simulink model "reinforcemen_model4"  (R2023b)
settings: Solver=FixedStepAuto  StartTime=0.0  StopTime=17  FixedStep=0.05  RelTol=1e-3  EnableMultiTasking=on
model workspace (MAT data in the model file):
  adjected_goal = 0
libraries: simulink x7, rllib x5
settings Model: SimulationMode=accelerator  ExtModeTrigDuration=2  Creator=MSI PC  LastModifiedBy=Yuk
settings SolverCC: AutoInsertRateTranBlk=on
settings OptimizationCC: DefaultParameterBehavior=Inlined  EnhancedBackFolding=on  PassReuseOutputArgsAs=Individual arguments  ZeroExternalMemoryAtStartup=off  ZeroInternalMemoryAtStartup=off  MaxStackSize=64  OptimizeBlockOrder=speed  DifferentSizesBufferReuse=on  OptimizationCustomize=off  EfficientTunableParamExpr=on
settings DebuggingCC: ParameterTunabilityLossMsg=error  UnconnectedInputMsg=warning  UnconnectedOutputMsg=warning  UnconnectedLineMsg=warning
settings HardwareCC: ProdBitPerPointer=32  ProdBitPerSizeT=32  ProdBitPerPtrDiffT=32  ProdLargestAtomicInteger=Long  ProdLargestAtomicFloat=Double  ProdWordSize=32  ProdHWDeviceType=ARM Compatible->ARM Cortex
settings ModelReferenceCC: EnableRefExpFcnMdlSchedulingChecks=on
settings SFSimCC: MATLABDynamicMemAlloc=off
settings RTWCC: Description=Embedded Coder  SystemTargetFile=ert.tlc  TemplateMakefile=ert_default_tmf  BuildConfiguration=Faster Runs  DLArmComputeVersion=19.05
settings CodeAppCC: ForceParamTrailComments=on  IgnoreCustomStorageClasses=off  OperatorAnnotations=on  SimulinkDataObjDesc=on  SFDataObjDesc=on  InsertBlockDesc=on
settings ERTTargetCC: SupportContinuousTime=on  SupportVariableSizeSignals=on  ExtModeTransport=3  ExtModeStaticAlloc=on  ExtModeAutomaticAllocSize=off  ExtModeStaticAllocSize=8192  ExtModeMexFile=ext_xcp  ExtModeIntrfLevel=Level2 - Open  ERTCustomFileTemplate=example_file_process.tlc

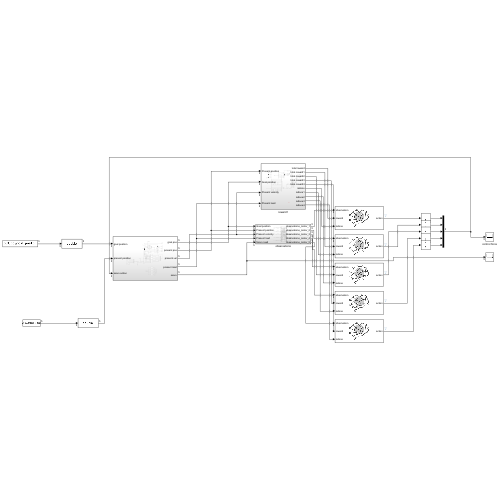
[thumbnail: Simulink's stored preview of the top-level diagram]
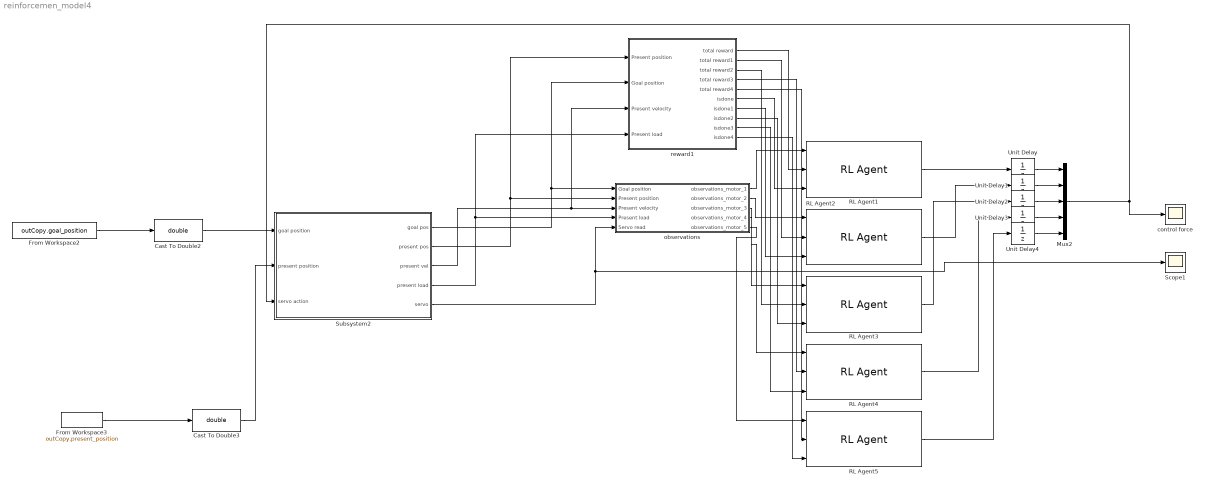
== system reinforcemen_model4 ==
  Cast To Double2 : DataTypeConversion  OutDataTypeStr=double  SaturateOnIntegerOverflow=off  RndMeth=Floor
  Cast To Double3 : DataTypeConversion  OutDataTypeStr=double  SaturateOnIntegerOverflow=off  RndMeth=Floor
  From Workspace2 : FromWorkspace  VariableName=outCopy.goal_position
  From Workspace3 : FromWorkspace  VariableName=outCopy.present_position
  Mux2 : Mux  Inputs=5
  RL Agent1 : rllib/RL Agent  Agent=agentA  ExternalActionAsInput=off  ProvideLastAction=off  ProvideCumRwd=off  TreatAsDirectFeedthrough=on  UseStrictObservationDataTypes=off
  RL Agent2 : rllib/RL Agent  Agent=agentB  ExternalActionAsInput=off  ProvideLastAction=off  ProvideCumRwd=off  TreatAsDirectFeedthrough=on  UseStrictObservationDataTypes=off
  RL Agent3 : rllib/RL Agent  Agent=agentC  ExternalActionAsInput=off  ProvideLastAction=off  ProvideCumRwd=off  TreatAsDirectFeedthrough=on  UseStrictObservationDataTypes=off
  RL Agent4 : rllib/RL Agent  Agent=agentD  ExternalActionAsInput=off  ProvideLastAction=off  ProvideCumRwd=off  TreatAsDirectFeedthrough=on  UseStrictObservationDataTypes=off
  RL Agent5 : rllib/RL Agent  Agent=agentE  ExternalActionAsInput=off  ProvideLastAction=off  ProvideCumRwd=off  TreatAsDirectFeedthrough=on  UseStrictObservationDataTypes=off
  Scope1 : Scope
  Subsystem2 : Subsystem
  Unit Delay : UnitDelay  SampleTime=-1  HasFrameUpgradeWarning=on
  Unit Delay{1..4} (4 alike) : UnitDelay  InitialCondition=180  SampleTime=-1  HasFrameUpgradeWarning=on
  control force : Scope
  observations : Subsystem
  reward1 : Subsystem
  wires:
  Subsystem2/1(goal pos) -> reward1/2(Goal position), observations/1(Goal position)
  RL Agent3/1 -> Unit Delay2/1
  RL Agent2/1 -> Unit Delay1/1
  RL Agent4/1 -> Unit Delay3/1
  RL Agent5/1 -> Unit Delay4/1
  observations/1(observations_motor_1) -> RL Agent1/1
  observations/2(observations_motor_2) -> RL Agent2/1
  observations/3(observations_motor_3) -> RL Agent3/1
  observations/4(observations_motor_4) -> RL Agent4/1
  observations/5(observations_motor_5) -> RL Agent5/1
  Subsystem2/5(servo) -> Scope1/1, observations/5(Servo read)
  reward1/1(total reward) -> RL Agent1/2
  reward1/2(total reward1) -> RL Agent2/2
  reward1/3(total reward2) -> RL Agent3/2
  reward1/4(total reward3) -> RL Agent4/2
  reward1/5(total reward4) -> RL Agent5/2
  reward1/6(isdone) -> RL Agent1/3
  reward1/7(isdone1) -> RL Agent2/3
  reward1/8(isdone2) -> RL Agent3/3
  reward1/9(isdone3) -> RL Agent4/3
  reward1/10(isdone4) -> RL Agent5/3
  Subsystem2/2(present pos) -> reward1/1(Present position), observations/2(Present position)
  Subsystem2/4(present load) -> reward1/4(Present load), observations/4(Present load)
  Subsystem2/3(present vel) -> reward1/3(Present velocity), observations/3(Present velocity)
  Mux2/1 -> Subsystem2/3(servo action), control force/1
  RL Agent1/1 -> Unit Delay/1
  Cast To Double2/1 -> Subsystem2/1(goal position)
  From Workspace2/1 -> Cast To Double2/1
  Cast To Double3/1 -> Subsystem2/2(present position)
  From Workspace3/1 -> Cast To Double3/1
  Unit Delay/1 -> Mux2/1
  Unit Delay1/1 -> Mux2/2
  Unit Delay2/1 -> Mux2/3
  Unit Delay3/1 -> Mux2/4
  Unit Delay4/1 -> Mux2/5

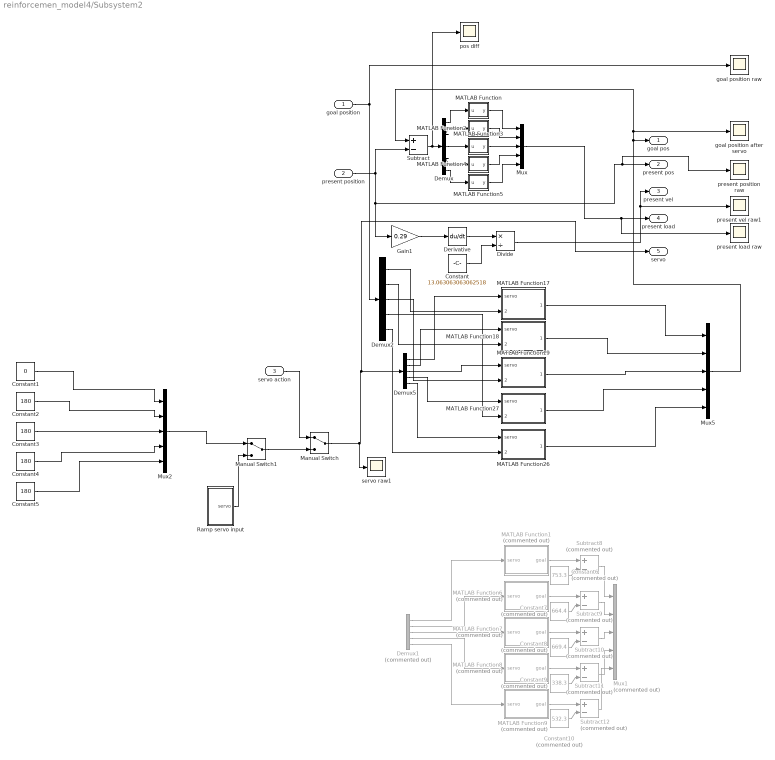
== system reinforcemen_model4/Subsystem2 ==
  goal position : Inport
  present position : Inport  Port=2
  servo action : Inport  Port=3
  Constant : Constant  Value=13.063063063062518
  Constant1 : Constant  Value=0
  Constant10 : Constant  Commented=on  Value=532.3
  Constant{2..5} (4 alike) : Constant  Value=180
  Constant6 : Constant  Commented=on  Value=753.3
  Constant7 : Constant  Commented=on  Value=664.4
  Constant8 : Constant  Commented=on  Value=669.4
  Constant9 : Constant  Commented=on  Value=338.3
  Demux : Demux  Outputs=5
  Demux1 : Demux  Commented=on  Outputs=5
  Demux2 : Demux  Outputs=5
  Demux5 : Demux  Outputs=5
  Derivative : Derivative
  Divide : Product  Inputs=*/
  Gain1 : Gain  Gain=0.29
  MATLAB Function : MATLAB Function  TreatAsAtomicUnit=on
  MATLAB Function1 : MATLAB Function  Commented=on  TreatAsAtomicUnit=on
  MATLAB Function17 : MATLAB Function  TreatAsAtomicUnit=on
  MATLAB Function18 : MATLAB Function  TreatAsAtomicUnit=on
  MATLAB Function19 : MATLAB Function  TreatAsAtomicUnit=on
  MATLAB Function2 : MATLAB Function  TreatAsAtomicUnit=on
  MATLAB Function26 : MATLAB Function  TreatAsAtomicUnit=on
  MATLAB Function27 : MATLAB Function  TreatAsAtomicUnit=on
  MATLAB Function3 : MATLAB Function  TreatAsAtomicUnit=on
  MATLAB Function4 : MATLAB Function  TreatAsAtomicUnit=on
  MATLAB Function5 : MATLAB Function  TreatAsAtomicUnit=on
  MATLAB Function6 : MATLAB Function  Commented=on  TreatAsAtomicUnit=on
  MATLAB Function7 : MATLAB Function  Commented=on  TreatAsAtomicUnit=on
  MATLAB Function8 : MATLAB Function  Commented=on  TreatAsAtomicUnit=on
  MATLAB Function9 : MATLAB Function  Commented=on  TreatAsAtomicUnit=on
  Manual Switch : ManualSwitch
  Manual Switch1 : ManualSwitch
  Mux : Mux  Inputs=5
  Mux1 : Mux  Commented=on  Inputs=5
  Mux2 : Mux  Inputs=5
  Mux5 : Mux  Inputs=5
  Ramp servo input : Subsystem
  Subtract : Sum  Inputs=+-
  Subtract{8..12} (5 alike) : Sum  Commented=on  Inputs=+-
  goal position after servo : Scope
  goal position raw : Scope
  pos diff : Scope
  present load raw : Scope
  present position raw : Scope
  present vel raw1 : Scope
  servo raw1 : Scope
  goal pos : Outport
  present pos : Outport  Port=2
  present vel : Outport  Port=3
  present load : Outport  Port=4
  servo : Outport  Port=5
  wires:
  goal position/1 -> goal position raw/1, Demux2/1
  present position/1 -> Subtract/2, Gain1/1, present position raw/1, present pos/1
  Demux/2 -> MATLAB Function2/1(u)
  MATLAB Function3/1(y) -> Mux/3
  Mux/1 -> present load raw/1, present load/1
  MATLAB Function/1(y) -> Mux/1
  MATLAB Function5/1(y) -> Mux/5
  MATLAB Function4/1(y) -> Mux/4
  Demux/4 -> MATLAB Function4/1(u)
  Demux/3 -> MATLAB Function3/1(u)
  Demux/1 -> MATLAB Function/1(u)
  Demux/5 -> MATLAB Function5/1(u)
  MATLAB Function2/1(y) -> Mux/2
  Constant/1 -> Divide/2
  Gain1/1 -> Derivative/1
  Derivative/1 -> Divide/1
  Divide/1 -> present vel raw1/1, present vel/1
  Demux5/3 -> MATLAB Function19/1(servo)
  Demux5/2 -> MATLAB Function18/1(servo)
  Demux5/1 -> MATLAB Function17/1(servo)
  Demux5/5 -> MATLAB Function26/1(servo)
  Demux5/4 -> MATLAB Function27/1(servo)
  Mux5/1 -> Subtract/1, goal position after servo/1, goal pos/1
  MATLAB Function9/1(goal) -> Subtract12/1
  Constant10/1 -> Subtract12/2
  Constant9/1 -> Subtract11/2
  MATLAB Function8/1(goal) -> Subtract11/1
  Subtract12/1 -> Mux1/5
  Subtract11/1 -> Mux1/4
  Subtract10/1 -> Mux1/3
  MATLAB Function7/1(goal) -> Subtract10/1
  Constant8/1 -> Subtract10/2
  Constant7/1 -> Subtract9/2
  Subtract9/1 -> Mux1/2
  Subtract8/1 -> Mux1/1
  MATLAB Function6/1(goal) -> Subtract9/1
  Constant6/1 -> Subtract8/2
  MATLAB Function1/1(goal) -> Subtract8/1
  Demux1/4 -> MATLAB Function8/1(servo)
  Demux1/5 -> MATLAB Function9/1(servo)
  Demux1/1 -> MATLAB Function1/1(servo)
  Demux1/2 -> MATLAB Function6/1(servo)
  Demux1/3 -> MATLAB Function7/1(servo)
  MATLAB Function17/1(adjected_goal) -> Mux5/1
  MATLAB Function18/1(adjected_goal) -> Mux5/2
  MATLAB Function19/1(adjected_goal) -> Mux5/3
  MATLAB Function27/1(adjected_goal) -> Mux5/4
  MATLAB Function26/1(adjected_goal) -> Mux5/5
  Constant2/1 -> Mux2/2
  Constant5/1 -> Mux2/5
  Constant1/1 -> Mux2/1
  Constant3/1 -> Mux2/3
  Constant4/1 -> Mux2/4
  Demux2/1 -> MATLAB Function17/2(init_goal)
  Demux2/2 -> MATLAB Function18/2(init_goal)
  Demux2/3 -> MATLAB Function19/2(init_goal)
  Demux2/4 -> MATLAB Function27/2(init_goal)
  Demux2/5 -> MATLAB Function26/2(init_goal)
  Manual Switch/1 -> servo raw1/1, servo/1, Demux5/1
  servo action/1 -> Manual Switch/1
  Manual Switch1/1 -> Manual Switch/2
  Mux2/1 -> Manual Switch1/1
  Ramp servo input/1(servo) -> Manual Switch1/2
  Subtract/1 -> pos diff/1, Demux/1

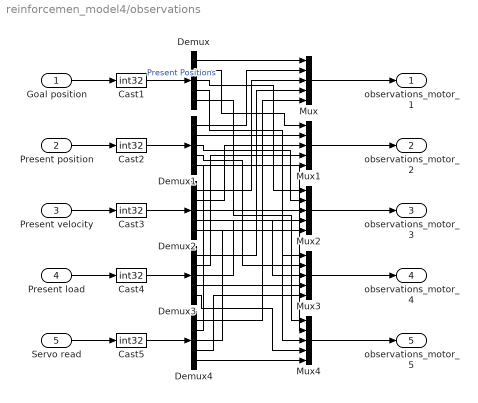
== system reinforcemen_model4/observations ==
  Goal position : Inport
  Present position : Inport  Port=2
  Present velocity : Inport  Port=3
  Present load : Inport  Port=4
  Servo read : Inport  Port=5
  Cast{1..5} (5 alike) : DataTypeConversion  OutDataTypeStr=int32  SaturateOnIntegerOverflow=off  RndMeth=Floor
  Demux{,1..4} (5 alike) : Demux  Outputs=5
  Mux{,1..4} (5 alike) : Mux  Inputs=5
  observations_motor_1 : Outport
  observations_motor_2 : Outport  Port=2
  observations_motor_3 : Outport  Port=3
  observations_motor_4 : Outport  Port=4
  observations_motor_5 : Outport  Port=5
  wires:
  Goal position/1 -> Cast1/1
  Present position/1 -> Cast2/1
  Present velocity/1 -> Cast3/1
  Present load/1 -> Cast4/1
  Servo read/1 -> Cast5/1
  Demux/1 -> Mux/1
  Demux1/1 -> Mux/2
  Demux2/1 -> Mux/3
  Demux3/1 -> Mux/4
  Demux4/1 -> Mux/5
  Demux/2 -> Mux1/1
  Demux1/2 -> Mux1/2
  Demux2/2 -> Mux1/3
  Demux3/2 -> Mux1/4
  Demux4/2 -> Mux1/5
  Demux/3 -> Mux2/1
  Demux1/3 -> Mux2/2
  Demux2/3 -> Mux2/3
  Demux3/3 -> Mux2/4
  Demux4/3 -> Mux2/5
  Demux/4 -> Mux3/1
  Demux1/4 -> Mux3/2
  Demux2/4 -> Mux3/3
  Demux3/4 -> Mux3/4
  Demux4/4 -> Mux3/5
  Demux/5 -> Mux4/1
  Demux1/5 -> Mux4/2
  Demux2/5 -> Mux4/3
  Demux3/5 -> Mux4/4
  Demux4/5 -> Mux4/5
  Mux/1 -> observations_motor_1/1
  Mux1/1 -> observations_motor_2/1
  Mux2/1 -> observations_motor_3/1
  Mux3/1 -> observations_motor_4/1
  Mux4/1 -> observations_motor_5/1
  Cast2/1 -> Demux1/1
  Cast3/1 -> Demux2/1
  Cast4/1 -> Demux3/1
  Cast5/1 -> Demux4/1
  Cast1/1 -> Demux/1  "Present Positions"

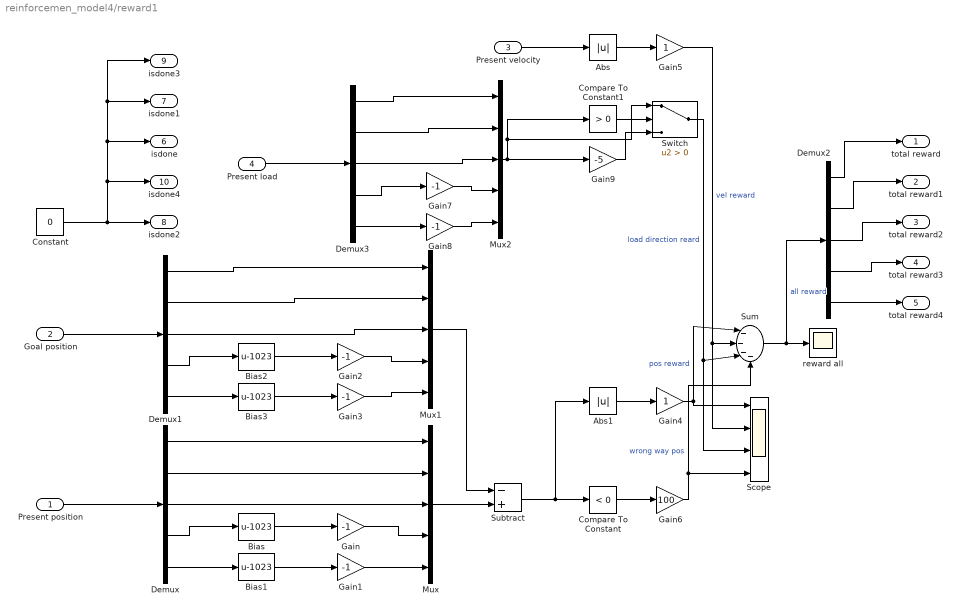
== system reinforcemen_model4/reward1 ==
  Present position : Inport
  Goal position : Inport  Port=2
  Present velocity : Inport  Port=3
  Present load : Inport  Port=4
  Abs : Abs  SaturateOnIntegerOverflow=off
  Abs1 : Abs  SaturateOnIntegerOverflow=off
  Bias{,1..3} (4 alike) : Bias  Bias=-1023  SaturateOnIntegerOverflow=off
  Compare To Constant : simulink/Logic and Bit Operations/Compare To Constant  relop=<  const=0  OutDataTypeStr=boolean
  Compare To Constant1 : simulink/Logic and Bit Operations/Compare To Constant  relop=>  const=0  OutDataTypeStr=boolean
  Constant : Constant  Value=0
  Demux{,1..3} (4 alike) : Demux  Outputs=5
  Gain{,1..3,7..8} (6 alike) : Gain  Gain=-1
  Gain4 : Gain
  Gain5 : Gain
  Gain6 : Gain  Gain=100
  Gain9 : Gain  Gain=-5
  Mux : Mux  Inputs=5
  Mux1 : Mux  Inputs=5
  Mux2 : Mux  Inputs=5
  Scope : Scope  NumInputPorts=4
  Subtract : Sum  Inputs=-+
  Sum : Sum  Inputs=|----
  Switch : Switch  Criteria=u2 > Threshold  SaturateOnIntegerOverflow=off  InputSameDT=off
  reward all : Scope
  total reward : Outport
  total reward1 : Outport  Port=2
  total reward2 : Outport  Port=3
  total reward3 : Outport  Port=4
  total reward4 : Outport  Port=5
  isdone : Outport  Port=6
  isdone1 : Outport  Port=7
  isdone2 : Outport  Port=8
  isdone3 : Outport  Port=9
  isdone4 : Outport  Port=10
  wires:
  Constant/1 -> isdone1/1, isdone3/1, isdone/1, isdone4/1, isdone2/1
  Abs1/1 -> Gain4/1
  Goal position/1 -> Demux1/1
  Demux/5 -> Bias1/1
  Present position/1 -> Demux/1
  Demux3/3 -> Mux2/3
  Demux1/3 -> Mux1/3
  Demux1/1 -> Mux1/1
  Demux1/2 -> Mux1/2
  Demux1/4 -> Bias2/1
  Bias/1 -> Gain/1
  Demux1/5 -> Bias3/1
  Demux/2 -> Mux/2
  Demux/1 -> Mux/1
  Bias3/1 -> Gain3/1
  Demux/3 -> Mux/3
  Bias1/1 -> Gain1/1
  Demux/4 -> Bias/1
  Mux2/1 -> Switch/1, Compare To Constant1/1, Gain9/1
  Gain4/1 -> Scope/1, Sum/1  "pos reward"
  Present load/1 -> Demux3/1
  Gain/1 -> Mux/4
  Bias2/1 -> Gain2/1
  Abs/1 -> Gain5/1
  Mux/1 -> Subtract/2
  Gain7/1 -> Mux2/4
  Demux3/1 -> Mux2/1
  Gain8/1 -> Mux2/5
  Demux3/2 -> Mux2/2
  Demux3/4 -> Gain7/1
  Demux3/5 -> Gain8/1
  Gain9/1 -> Switch/3
  Gain2/1 -> Mux1/4
  Compare To Constant1/1 -> Switch/2
  Gain3/1 -> Mux1/5
  Gain1/1 -> Mux/5
  Compare To Constant/1 -> Gain6/1
  Mux1/1 -> Subtract/1
  Switch/1 -> Sum/3, Scope/3  "load direction reard"
  Present velocity/1 -> Abs/1
  Subtract/1 -> Compare To Constant/1, Abs1/1
  ? -> ?  "control reward"
  Gain5/1 -> Sum/2, Scope/2  "vel reward"
  Gain6/1 -> Sum/4, Scope/4  "wrong way pos"
  Sum/1 -> reward all/1, Demux2/1  "all reward"
  Demux2/1 -> total reward/1
  Demux2/2 -> total reward1/1
  Demux2/3 -> total reward2/1
  Demux2/4 -> total reward3/1
  Demux2/5 -> total reward4/1

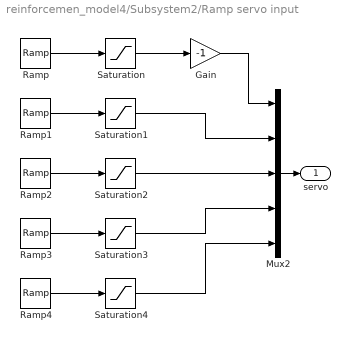
== system reinforcemen_model4/Subsystem2/Ramp servo input ==
  Gain : Gain  Gain=-1
  Mux2 : Mux  Inputs=5
  Ramp : simulink/Sources/Ramp  slope=25  start=1  InitialOutput=-125
  Ramp{1..4} (4 alike) : simulink/Sources/Ramp  slope=25  start=1  InitialOutput=70
  Saturation : Saturate  UpperLimit=0  LowerLimit=-125
  Saturation{1..4} (4 alike) : Saturate  UpperLimit=180  LowerLimit=70
  servo : Outport
  wires:
  Gain/1 -> Mux2/1
  Saturation2/1 -> Mux2/3
  Saturation3/1 -> Mux2/4
  Ramp3/1 -> Saturation3/1
  Saturation1/1 -> Mux2/2
  Ramp4/1 -> Saturation4/1
  Ramp/1 -> Saturation/1
  Saturation4/1 -> Mux2/5
  Ramp2/1 -> Saturation2/1
  Ramp1/1 -> Saturation1/1
  Saturation/1 -> Gain/1
  Mux2/1 -> servo/1

== matlab function reinforcemen_model4/Subsystem2/MATLAB Function8 ==
  data: servo input; goal output
function goal = nonlinearRegressionModel4(servo)
    % 학습된 모델 파라미터
    a = 1335; % 예시 값
    b = 129.9; % 예시 값
    c = -0.02157; % 예시 값
   

    % 비선형 회귀 모델을 이용한 로드 값 계산
    goal = a / (1 + exp(-c*(servo-b)));
end

== matlab function reinforcemen_model4/Subsystem2/MATLAB Function9 ==
  data: servo input; goal output
function goal = nonlinearRegressionModel5(servo)
    % 학습된 모델 파라미터
    a = 1134; % 예시 값
    b = 174.7; % 예시 값
    c = -0.02309; % 예시 값
   

    % 비선형 회귀 모델을 이용한 로드 값 계산
    goal = a / (1 + exp(-c*(servo-b)));
end

== matlab function reinforcemen_model4/Subsystem2/MATLAB Function1 ==
  data: servo input; goal output
function goal = nonlinearRegressionModel1(servo)
    % 학습된 모델 파라미터
    a = 756; % 예시 값
    b = 28.73; % 예시 값
    c = -0.1959; % 예시 값
   

    % 비선형 회귀 모델을 이용한 로드 값 계산
    goal = a / (1 + exp(-c*(servo-b)));
end

== matlab function reinforcemen_model4/Subsystem2/MATLAB Function17 ==
  data: servo input; adjected_goal output; init_goal input
function adjected_goal = nonlinearRegressionModel1(servo,init_goal)
    % 학습된 모델 파라미터
    a = 756; % 예시 값
    b = 28.73; % 예시 값
    c = -0.1959; % 예시 값
   
    adjected_goal = init_goal;
    
    bound = a / (1 + exp(-c*(servo-b)));
    if init_goal > bound
    adjected_goal = bound;
    else
        adjected_goal = init_goal;
    end


end

== matlab function reinforcemen_model4/Subsystem2/MATLAB Function18 ==
  data: servo input; adjected_goal output; init_goal input
function adjected_goal = nonlinearRegressionModel2(servo,init_goal)
    % 학습된 모델 파라미터
    a = 665.6; % 예시 값
    b = 121.3; % 예시 값
    c = 0.1082; % 예시 값
   
    adjected_goal = init_goal;
    % 비선형 회귀 모델을 이용한 로드 값 계산
    bound = a / (1 + exp(-c*(servo-b)));

    if init_goal > bound
        adjected_goal = bound;
    else
        adjected_goal = init_goal;
    end
end

== matlab function reinforcemen_model4/Subsystem2/MATLAB Function19 ==
  data: servo input; adjected_goal output; init_goal input
function adjected_goal = nonlinearRegressionModel3(servo,init_goal)
    % 학습된 모델 파라미터
    a = 669.4; % 예시 값
    b = 115.4; % 예시 값
    c = 0.1683; % 예시 값
   
    adjected_goal = init_goal;
    % 비선형 회귀 모델을 이용한 로드 값 계산
    bound = a / (1 + exp(-c*(servo-b)));

    if init_goal > bound
        adjected_goal = bound;
    else
        adjected_goal = init_goal;
    end
end

== matlab function reinforcemen_model4/Subsystem2/MATLAB Function2 ==
  data: u input; y output
function y = fcn(u)
    m = -0.6479; % 모델의 기울기
    b = -2.7392; % y절편
    y = m * u + b; % 선형 회귀 모델의 계산

    if y >=100
        y = 100;
    elseif y <=-100
        y = -100;
    else
        y = y;
    end
end

== matlab function reinforcemen_model4/Subsystem2/MATLAB Function26 ==
  data: servo input; adjected_goal output; init_goal input
function adjected_goal = nonlinearRegressionModel5(servo,init_goal)
    % 학습된 모델 파라미터
    a = 672.4; % 예시 값
    b = 127; % 예시 값
    c = 0.07872; % 예시 값
    adjected_goal = init_goal;

    % 비선형 회귀 모델을 이용한 로드 값 계산
    bound = -(a / (1 + exp(-c*(servo-b))))+1023;

    if init_goal < bound
        adjected_goal = bound;
    else
        adjected_goal = init_goal;
    end
end

== matlab function reinforcemen_model4/Subsystem2/MATLAB Function27 ==
  data: servo input; adjected_goal output; init_goal input
function adjected_goal = nonlinearRegressionModel4(servo,init_goal)
    % 학습된 모델 파라미터
    a = 678.9; % 예시 값
    b = 138.5; % 예시 값
    c = 0.1073; % 예시 값
   
    adjected_goal = init_goal;
    % 비선형 회귀 모델을 이용한 로드 값 계산
    bound = - (a / (1 + exp(-c*(servo-b))))+1023;

    if init_goal < bound
        adjected_goal = bound;
    else
        adjected_goal = init_goal;
    end
end

== matlab function reinforcemen_model4/Subsystem2/MATLAB Function3 ==
  data: u input; y output
function y = fcn(u)
    m = -0.6455; % 모델의 기울기
    b = -3.7139; % y절편
    y = m * u + b; % 선형 회귀 모델의 계산


    if y >=100
        y = 100;
    elseif y <=-100
        y = -100;
    else
        y = y;
    end
end

== matlab function reinforcemen_model4/Subsystem2/MATLAB Function4 ==
  data: u input; y output
function y = fcn(u)
    m = -0.7081; % 모델의 기울기
    b = 2.9215; % y절편
    y = m * u + b; % 선형 회귀 모델의 계산

    if y >=100
        y = 100;
    elseif y <=-100
        y = -100;
    else
        y = y;
    end
end

== matlab function reinforcemen_model4/Subsystem2/MATLAB Function5 ==
  data: u input; y output
function y = fcn(u)
    m = -0.6317; % 모델의 기울기
    b = 2.8366; % y절편
    y = m * u + b; % 선형 회귀 모델의 계산

    if y >=100
        y = 100;
    elseif y <=-100
        y = -100;
    else
        y = y;
    end
end

== matlab function reinforcemen_model4/Subsystem2/MATLAB Function ==
  data: u input; y output
function y = fcn(u)
    m = -0.5989; % 모델의 기울기
    b = -5.1558; % y절편
    y = m * u + b; % 선형 회귀 모델의 계산

    if y >=100
        y = 100;
    elseif y <=-100
        y = -100;
    else
        y = y;
    end
end

== matlab function reinforcemen_model4/Subsystem2/MATLAB Function6 ==
  data: servo input; goal output
function goal = nonlinearRegressionModel2(servo)
    % 학습된 모델 파라미터
    a = 665.6; % 예시 값
    b = 121.3; % 예시 값
    c = 0.1082; % 예시 값
   

    % 비선형 회귀 모델을 이용한 로드 값 계산
    goal = a / (1 + exp(-c*(servo-b)));
end

== matlab function reinforcemen_model4/Subsystem2/MATLAB Function7 ==
  data: servo input; goal output
function goal = nonlinearRegressionModel3(servo)
    % 학습된 모델 파라미터
    a = 669.4; % 예시 값
    b = 115.4; % 예시 값
    c = 0.1683; % 예시 값
   

    % 비선형 회귀 모델을 이용한 로드 값 계산
    goal = a / (1 + exp(-c*(servo-b)));
end
